simulink model "pid_board"  (R2024b)
settings: Solver=ode4  StartTime=0.0  StopTime=10.0  FixedStep=pcb.sim_dt  RelTol=1e-3
PostLoadFcn:
  | pbdir_ = fileparts(get_param('pid_board', 'FileName')); if ~exist('pcb', 'var'), run(fullfile(pbdir_, 'pid_board_params.m')); end; if ~exist('CtrlIn', 'var'), run(fullfile(pbdir_, '..', 'common', 'quad_ctrl_buses.m')); end; clear pbdir_
model workspace (MAT data in the model file):
  board_variant = Simulink.Parameter
  board_variant.Value = 1
  board_variant.Complexity = 'real'
  board_variant.Dimensions = [1 1]
  board_variant.Description = 'Analog section: 1 = pid_analog_fast, 2 = pid_analog_circuit'
  board_variant.DataType = 'double'
values from neighbouring files (symbols this model uses):
  pcb = evalin('base', 'pcb')    [pid_analog_circuit_test.m]    (also in pid_board_bench_inputs.m; pid_board_params.m = struct(); pid_board_validate.m)
Description:
  | PID_Board rev B digital twin (Model 2, fast). ctrl_in (CtrlIn bus) -> shim U1 -> DACs -> analog section (variant pcb.variant) -> control_io U3 -> esc_us [M1 RR, M2 FR, M3 RL, M4 FL].
settings Model: ParameterArgumentNames=board_variant  Creator=doubi  LastModifiedBy=doubi

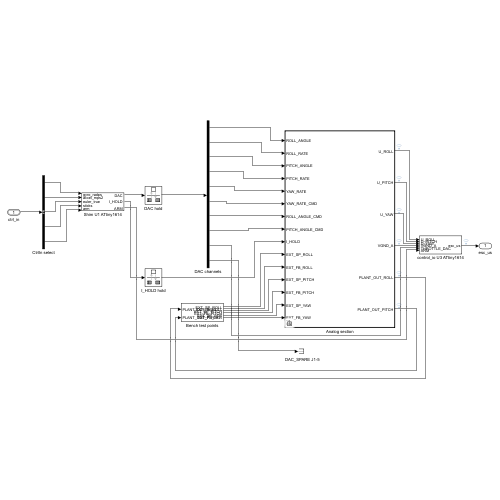
[thumbnail: Simulink's stored preview of the top-level diagram]
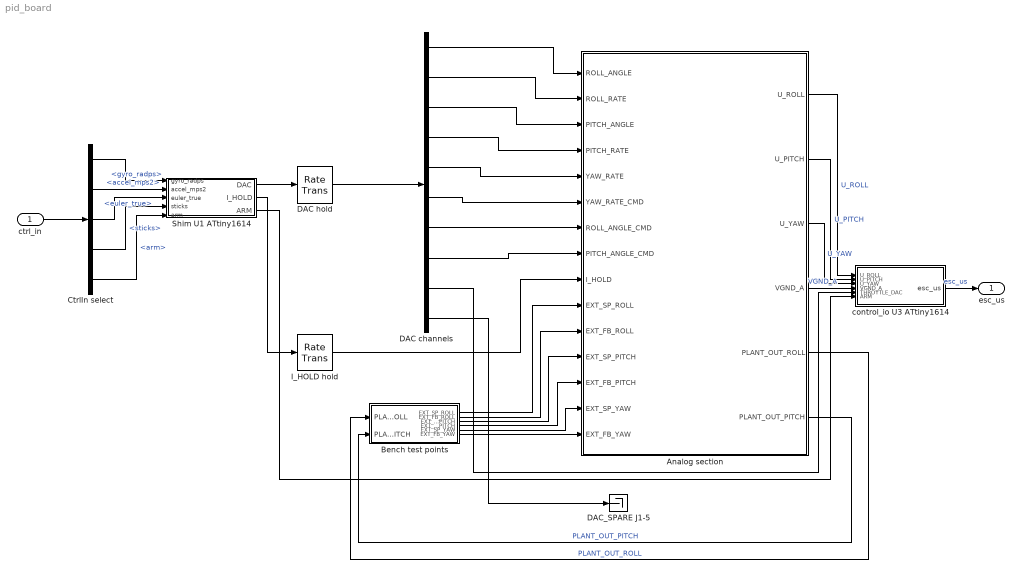
== system pid_board ==
  ctrl_in : Inport  OutDataTypeStr=Bus: CtrlIn  SampleTime=1e-3
  Analog section : Subsystem  Variant=on  VariantActivationTime=startup
  Bench test points : Subsystem  mask{brd=pcb}
      mask init:
      | w1p = [brd.VG + brd.bench.w1_offset, brd.bench.w1_amp, brd.bench.w1_freq, brd.bench.w1_t0];
  CtrlIn select : BusSelector  OutputSignals=gyro_radps,accel_mps2,euler_true,sticks,arm
  DAC channels : Demux  Outputs=10
  DAC hold : RateTransition  OutPortSampleTime=0
  DAC_SPARE J1-5 : Terminator
  I_HOLD hold : RateTransition  OutPortSampleTime=0
  Shim U1 ATtiny1614 : Subsystem  mask{brd=pcb}
      mask init:
      | Ts = brd.shim.Ts; g0 = 9.80665;
      | shp = [brd.shim.Ts, brd.shim.cf_alpha, brd.shim.axis_sign(:).', brd.shim.angle_src, brd.scale.Kw, brd.scale.Ktheta, brd.shim.angle_max, brd.shim.yaw_rate_max, brd.scale.thr_V0, brd.scale.thr_V1, brd.shim.ihold_low_thr, brd.shim.thr_low, brd.ihold.t_release, brd.VG];
      | crp = [brd.shim.crsf_min, brd.shim.crsf_mid, brd.shim.crsf_max];
      | nstd = brd.shim.noise_on*brd.shim.gyro_nd*sqrt(1/(2*brd.shim.Ts));
  control_io U3 ATtiny1614 : Subsystem  mask{brd=pcb}
      mask init:
      | Ts = brd.ctrl.Ts;
      | cp = [brd.ctrl.adc_lsb, brd.ctrl.adc_bits, brd.scale.thr_V0, brd.scale.thr_V1, brd.ctrl.us_off, brd.ctrl.us_idle, brd.ctrl.us_max, brd.ctrl.us_res, brd.ctrl.K_rpy(:).'];
      | mixm = brd.ctrl.mix;
  esc_us : Outport
  wires:
  ctrl_in/1 -> CtrlIn select/1
  CtrlIn select/2 -> Shim U1 ATtiny1614/2(accel_mps2)  "<accel_mps2>"
  CtrlIn select/4 -> Shim U1 ATtiny1614/4(sticks)  "<sticks>"
  Shim U1 ATtiny1614/2(I_HOLD) -> I_HOLD hold/1
  CtrlIn select/1 -> Shim U1 ATtiny1614/1(gyro_radps)  "<gyro_radps>"
  CtrlIn select/3 -> Shim U1 ATtiny1614/3(euler_true)  "<euler_true>"
  CtrlIn select/5 -> Shim U1 ATtiny1614/5(arm)  "<arm>"
  Bench test points/1(EXT_SP_ROLL) -> Analog section/10(EXT_SP_ROLL)
  Shim U1 ATtiny1614/1(DAC) -> DAC hold/1
  Shim U1 ATtiny1614/3(ARM) -> control_io U3 ATtiny1614/6(ARM)
  control_io U3 ATtiny1614/1(esc_us) -> esc_us/1  "esc_us"
  Analog section/4(VGND_A) -> control_io U3 ATtiny1614/4(VGND_A)  "VGND_A"
  DAC hold/1 -> DAC channels/1
  DAC channels/6 -> Analog section/6(YAW_RATE_CMD)
  I_HOLD hold/1 -> Analog section/9(I_HOLD)
  DAC channels/1 -> Analog section/1(ROLL_ANGLE)
  DAC channels/2 -> Analog section/2(ROLL_RATE)
  DAC channels/3 -> Analog section/3(PITCH_ANGLE)
  DAC channels/4 -> Analog section/4(PITCH_RATE)
  DAC channels/5 -> Analog section/5(YAW_RATE)
  DAC channels/7 -> Analog section/7(ROLL_ANGLE_CMD)
  Analog section/5(PLANT_OUT_ROLL) -> Bench test points/1(PLANT_OUT_ROLL)  "PLANT_OUT_ROLL"
  DAC channels/8 -> Analog section/8(PITCH_ANGLE_CMD)
  Analog section/6(PLANT_OUT_PITCH) -> Bench test points/2(PLANT_OUT_PITCH)  "PLANT_OUT_PITCH"
  DAC channels/9 -> control_io U3 ATtiny1614/5(THROTTLE_DAC)
  Analog section/3(U_YAW) -> control_io U3 ATtiny1614/3(U_YAW)  "U_YAW"
  DAC channels/10 -> DAC_SPARE J1-5/1
  Bench test points/2(EXT_FB_ROLL) -> Analog section/11(EXT_FB_ROLL)
  Bench test points/3(EXT_SP_PITCH) -> Analog section/12(EXT_SP_PITCH)
  Bench test points/4(EXT_FB_PITCH) -> Analog section/13(EXT_FB_PITCH)
  Bench test points/5(EXT_SP_YAW) -> Analog section/14(EXT_SP_YAW)
  Bench test points/6(EXT_FB_YAW) -> Analog section/15(EXT_FB_YAW)
  Analog section/1(U_ROLL) -> control_io U3 ATtiny1614/1(U_ROLL)  "U_ROLL"
  Analog section/2(U_PITCH) -> control_io U3 ATtiny1614/2(U_PITCH)  "U_PITCH"

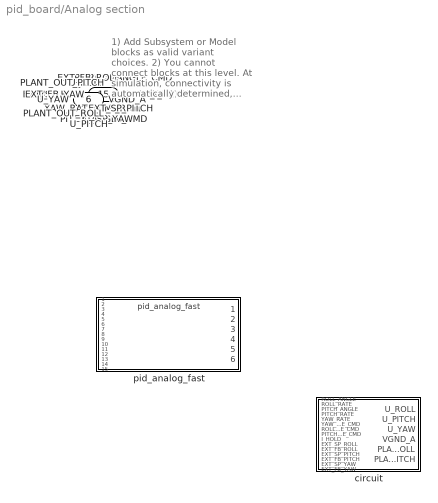
== system pid_board/Analog section ==
  note: 1) Add Subsystem or Model blocks as valid variant choices.
      | 2) You cannot connect blocks at this level. At simulation, connectivity is automatically
      | determined, based on the active variant and port name matching.
  ROLL_ANGLE : Inport
  ROLL_RATE : Inport  Port=2
  PITCH_ANGLE : Inport  Port=3
  PITCH_RATE : Inport  Port=4
  YAW_RATE : Inport  Port=5
  YAW_RATE_CMD : Inport  Port=6
  ROLL_ANGLE_CMD : Inport  Port=7
  PITCH_ANGLE_CMD : Inport  Port=8
  I_HOLD : Inport  Port=9
  EXT_SP_ROLL : Inport  Port=10
  EXT_FB_ROLL : Inport  Port=11
  EXT_SP_PITCH : Inport  Port=12
  EXT_FB_PITCH : Inport  Port=13
  EXT_SP_YAW : Inport  Port=14
  EXT_FB_YAW : Inport  Port=15
  circuit : Subsystem  TreatAsAtomicUnit=on  Variant=on  VariantControl=board_variant == 2  AllowZeroVariantControls=on
  pid_analog_fast : ModelReference  ModelNameDialog=pid_analog_fast  SimulationMode=Normal  VariantControl=board_variant == 1  ModelReferenceVersion=1.1
  U_ROLL : Outport
  U_PITCH : Outport  Port=2
  U_YAW : Outport  Port=3
  VGND_A : Outport  Port=4
  PLANT_OUT_ROLL : Outport  Port=5
  PLANT_OUT_PITCH : Outport  Port=6

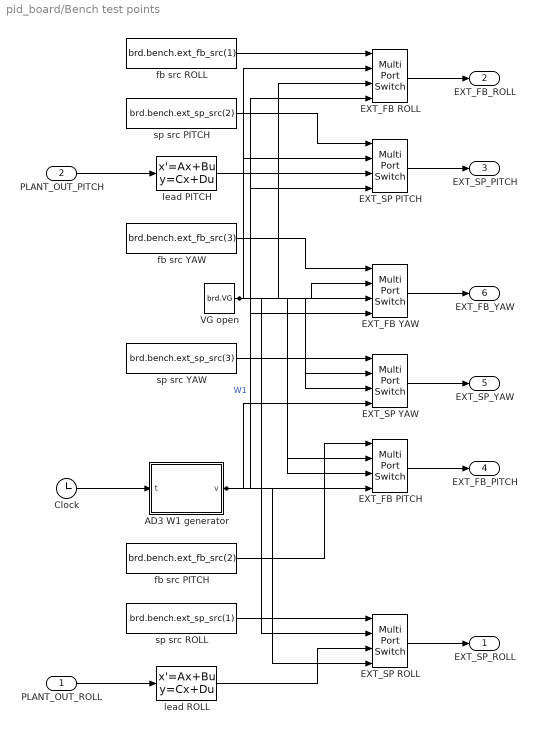
== system pid_board/Bench test points ==
  PLANT_OUT_ROLL : Inport
  PLANT_OUT_PITCH : Inport  Port=2
  AD3 W1 generator : MATLAB Function  TreatAsAtomicUnit=on
  Clock : Clock
  EXT_FB PITCH : MultiPortSwitch  DataPortOrder=Zero-based contiguous  zeroidx=on  SaturateOnIntegerOverflow=off  InputSameDT=off
  EXT_FB ROLL : MultiPortSwitch  DataPortOrder=Zero-based contiguous  zeroidx=on  SaturateOnIntegerOverflow=off  InputSameDT=off
  EXT_FB YAW : MultiPortSwitch  DataPortOrder=Zero-based contiguous  zeroidx=on  SaturateOnIntegerOverflow=off  InputSameDT=off
  EXT_SP PITCH : MultiPortSwitch  DataPortOrder=Zero-based contiguous  zeroidx=on  SaturateOnIntegerOverflow=off  InputSameDT=off
  EXT_SP ROLL : MultiPortSwitch  DataPortOrder=Zero-based contiguous  zeroidx=on  SaturateOnIntegerOverflow=off  InputSameDT=off
  EXT_SP YAW : MultiPortSwitch  DataPortOrder=Zero-based contiguous  zeroidx=on  SaturateOnIntegerOverflow=off  InputSameDT=off
  VG open : Constant  Value=brd.VG  SampleTime=0
  fb src PITCH : Constant  Value=brd.bench.ext_fb_src(2)
  fb src ROLL : Constant  Value=brd.bench.ext_fb_src(1)
  fb src YAW : Constant  Value=brd.bench.ext_fb_src(3)
  lead PITCH : StateSpace  A=-1/brd.bench.lead_tau  B=1/brd.bench.lead_tau  D=0  InitialCondition=brd.VG
  lead ROLL : StateSpace  A=-1/brd.bench.lead_tau  B=1/brd.bench.lead_tau  D=0  InitialCondition=brd.VG
  sp src PITCH : Constant  Value=brd.bench.ext_sp_src(2)
  sp src ROLL : Constant  Value=brd.bench.ext_sp_src(1)
  sp src YAW : Constant  Value=brd.bench.ext_sp_src(3)
  EXT_SP_ROLL : Outport
  EXT_FB_ROLL : Outport  Port=2
  EXT_SP_PITCH : Outport  Port=3
  EXT_FB_PITCH : Outport  Port=4
  EXT_SP_YAW : Outport  Port=5
  EXT_FB_YAW : Outport  Port=6
  wires:
  PLANT_OUT_PITCH/1 -> lead PITCH/1
  VG open/1 -> EXT_SP ROLL/2, EXT_FB ROLL/2, EXT_FB PITCH/2, EXT_FB ROLL/3, EXT_SP YAW/2, EXT_SP YAW/3, EXT_SP PITCH/2, EXT_FB YAW/2, EXT_FB PITCH/3, EXT_FB YAW/3
  Clock/1 -> AD3 W1 generator/1(t)
  PLANT_OUT_ROLL/1 -> lead ROLL/1
  lead PITCH/1 -> EXT_SP PITCH/3
  sp src PITCH/1 -> EXT_SP PITCH/1
  fb src ROLL/1 -> EXT_FB ROLL/1
  fb src YAW/1 -> EXT_FB YAW/1
  EXT_SP YAW/1 -> EXT_SP_YAW/1
  sp src YAW/1 -> EXT_SP YAW/1
  AD3 W1 generator/1(v) -> EXT_SP ROLL/4, EXT_FB ROLL/4, EXT_FB PITCH/4, EXT_SP PITCH/4, EXT_SP YAW/4, EXT_FB YAW/4  "W1"
  EXT_FB ROLL/1 -> EXT_FB_ROLL/1
  fb src PITCH/1 -> EXT_FB PITCH/1
  sp src ROLL/1 -> EXT_SP ROLL/1
  lead ROLL/1 -> EXT_SP ROLL/3
  EXT_SP PITCH/1 -> EXT_SP_PITCH/1
  EXT_FB YAW/1 -> EXT_FB_YAW/1
  EXT_FB PITCH/1 -> EXT_FB_PITCH/1
  EXT_SP ROLL/1 -> EXT_SP_ROLL/1

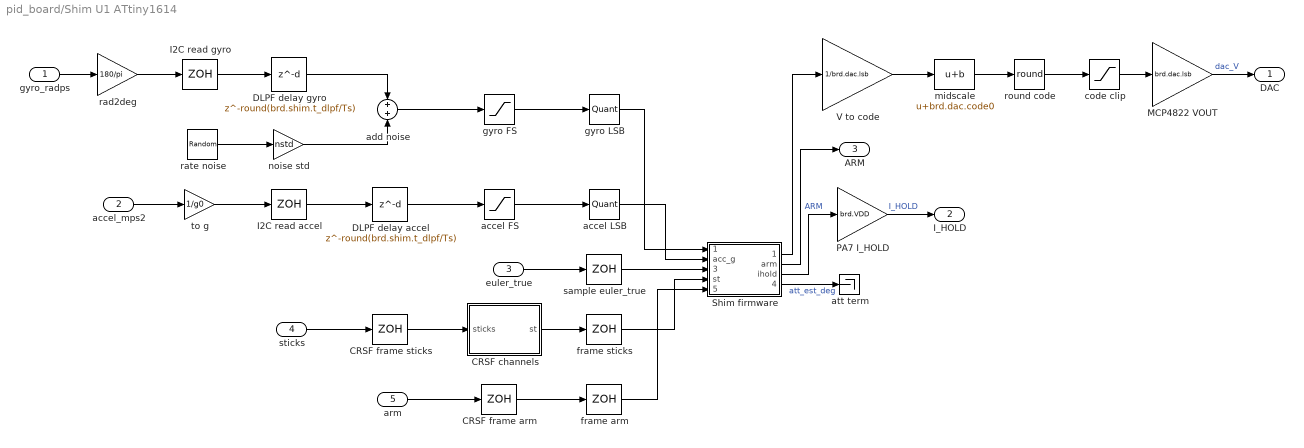
== system pid_board/Shim U1 ATtiny1614 ==
  gyro_radps : Inport
  accel_mps2 : Inport  Port=2
  euler_true : Inport  Port=3
  sticks : Inport  Port=4
  arm : Inport  Port=5
  CRSF channels : MATLAB Function  TreatAsAtomicUnit=on
  CRSF frame arm : ZeroOrderHold  SampleTime=brd.shim.crsf_Ts
  CRSF frame sticks : ZeroOrderHold  SampleTime=brd.shim.crsf_Ts
  DLPF delay accel : Delay  DelayLength=round(brd.shim.t_dlpf/Ts)
  DLPF delay gyro : Delay  DelayLength=round(brd.shim.t_dlpf/Ts)
  I2C read accel : ZeroOrderHold  SampleTime=Ts
  I2C read gyro : ZeroOrderHold  SampleTime=Ts
  MCP4822 VOUT : Gain  Gain=brd.dac.lsb
  PA7 I_HOLD : Gain  Gain=brd.VDD
  Shim firmware : MATLAB Function  TreatAsAtomicUnit=on
  V to code : Gain  Gain=1/brd.dac.lsb
  accel FS : Saturate  UpperLimit=brd.shim.acc_fs  LowerLimit=-brd.shim.acc_fs
  accel LSB : Quantizer  QuantizationInterval=brd.shim.acc_lsb
  add noise : Sum
  att term : Terminator
  code clip : Saturate  UpperLimit=2^brd.dac.bits - 1  LowerLimit=0
  frame arm : ZeroOrderHold  SampleTime=Ts
  frame sticks : ZeroOrderHold  SampleTime=Ts
  gyro FS : Saturate  UpperLimit=brd.shim.gyro_fs  LowerLimit=-brd.shim.gyro_fs
  gyro LSB : Quantizer  QuantizationInterval=brd.shim.gyro_lsb
  midscale : Bias  Bias=brd.dac.code0  SaturateOnIntegerOverflow=off
  noise std : Gain  Gain=nstd
  rad2deg : Gain  Gain=180/pi
  rate noise : RandomNumber  Mean=[0 0 0]  Variance=[1 1 1]  Seed=[23341 23342 23343]  SampleTime=Ts
  round code : Rounding  Operator=round
  sample euler_true : ZeroOrderHold  SampleTime=Ts
  to g : Gain  Gain=1/g0
  DAC : Outport
  I_HOLD : Outport  Port=2
  ARM : Outport  Port=3
  wires:
  gyro_radps/1 -> rad2deg/1
  noise std/1 -> add noise/2
  I2C read gyro/1 -> DLPF delay gyro/1
  rate noise/1 -> noise std/1
  frame arm/1 -> Shim firmware/5(arm_in)
  rad2deg/1 -> I2C read gyro/1
  euler_true/1 -> sample euler_true/1
  to g/1 -> I2C read accel/1
  accel FS/1 -> accel LSB/1
  accel_mps2/1 -> to g/1
  frame sticks/1 -> Shim firmware/4(st)
  DLPF delay gyro/1 -> add noise/1
  I2C read accel/1 -> DLPF delay accel/1
  sticks/1 -> CRSF frame sticks/1
  add noise/1 -> gyro FS/1
  PA7 I_HOLD/1 -> I_HOLD/1  "I_HOLD"
  accel LSB/1 -> Shim firmware/2(acc_g)
  DLPF delay accel/1 -> accel FS/1
  sample euler_true/1 -> Shim firmware/3(euler_rad)
  CRSF frame sticks/1 -> CRSF channels/1(sticks)
  arm/1 -> CRSF frame arm/1
  gyro FS/1 -> gyro LSB/1
  CRSF channels/1(st) -> frame sticks/1
  CRSF frame arm/1 -> frame arm/1
  gyro LSB/1 -> Shim firmware/1(gyro_dps)
  Shim firmware/1(dac_rel) -> V to code/1
  Shim firmware/2(arm) -> ARM/1  "ARM"
  midscale/1 -> round code/1
  Shim firmware/3(ihold) -> PA7 I_HOLD/1
  Shim firmware/4(att_deg) -> att term/1  "att_est_deg"
  V to code/1 -> midscale/1
  round code/1 -> code clip/1
  code clip/1 -> MCP4822 VOUT/1
  MCP4822 VOUT/1 -> DAC/1  "dac_V"

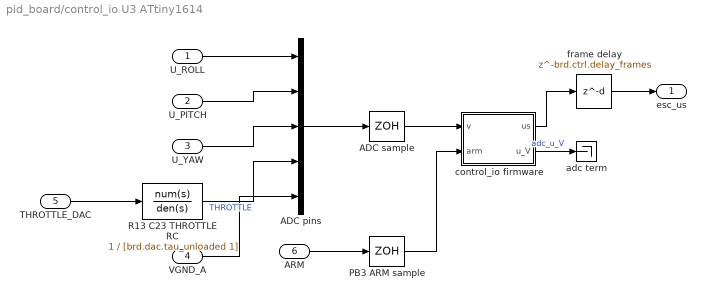
== system pid_board/control_io U3 ATtiny1614 ==
  U_ROLL : Inport
  U_PITCH : Inport  Port=2
  U_YAW : Inport  Port=3
  VGND_A : Inport  Port=4
  THROTTLE_DAC : Inport  Port=5
  ARM : Inport  Port=6
  ADC pins : Mux  Inputs=5
  ADC sample : ZeroOrderHold  SampleTime=Ts
  PB3 ARM sample : ZeroOrderHold  SampleTime=Ts
  R13 C23 THROTTLE RC : TransferFcn  Numerator=1  Denominator=[brd.dac.tau_unloaded 1]
  adc term : Terminator
  control_io firmware : MATLAB Function  TreatAsAtomicUnit=on
  frame delay : Delay  DelayLength=brd.ctrl.delay_frames  InitialCondition=brd.ctrl.us_off
  esc_us : Outport
  wires:
  U_YAW/1 -> ADC pins/3
  THROTTLE_DAC/1 -> R13 C23 THROTTLE RC/1
  U_ROLL/1 -> ADC pins/1
  ARM/1 -> PB3 ARM sample/1
  ADC pins/1 -> ADC sample/1
  R13 C23 THROTTLE RC/1 -> ADC pins/4  "THROTTLE"
  VGND_A/1 -> ADC pins/5
  U_PITCH/1 -> ADC pins/2
  ADC sample/1 -> control_io firmware/1(v)
  control_io firmware/1(us) -> frame delay/1
  PB3 ARM sample/1 -> control_io firmware/2(arm)
  control_io firmware/2(u_V) -> adc term/1  "adc_u_V"
  frame delay/1 -> esc_us/1

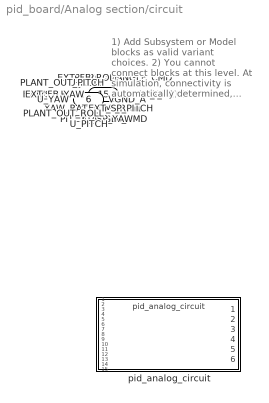
== system pid_board/Analog section/circuit ==
  note: 1) Add Subsystem or Model blocks as valid variant choices.
      | 2) You cannot connect blocks at this level. At simulation, connectivity is automatically
      | determined, based on the active variant and port name matching.
  ROLL_ANGLE : Inport
  ROLL_RATE : Inport  Port=2
  PITCH_ANGLE : Inport  Port=3
  PITCH_RATE : Inport  Port=4
  YAW_RATE : Inport  Port=5
  YAW_RATE_CMD : Inport  Port=6
  ROLL_ANGLE_CMD : Inport  Port=7
  PITCH_ANGLE_CMD : Inport  Port=8
  I_HOLD : Inport  Port=9
  EXT_SP_ROLL : Inport  Port=10
  EXT_FB_ROLL : Inport  Port=11
  EXT_SP_PITCH : Inport  Port=12
  EXT_FB_PITCH : Inport  Port=13
  EXT_SP_YAW : Inport  Port=14
  EXT_FB_YAW : Inport  Port=15
  pid_analog_circuit : ModelReference  ModelNameDialog=pid_analog_circuit  SimulationMode=Normal  VariantControl=pcb.circuit_enable == 1  ModelReferenceVersion=1.10
  U_ROLL : Outport
  U_PITCH : Outport  Port=2
  U_YAW : Outport  Port=3
  VGND_A : Outport  Port=4
  PLANT_OUT_ROLL : Outport  Port=5
  PLANT_OUT_PITCH : Outport  Port=6

== matlab function pid_board/Shim U1 ATtiny1614/Shim firmware ==
  data: gyro_dps input size=[3 1]; dac_rel output size=[10 1]; acc_g input size=[3 1]; euler_rad input size=[3 1]; st input size=[4 1]; arm_in input size=1; arm output size=1; ihold output size=1; att_deg output size=[2 1]; shp parameter
function [dac_rel, arm, ihold, att_deg] = shim_fw(gyro_dps, acc_g, euler_rad, st, arm_in, shp)
%Shim U1 firmware model (ASSUMED behaviour, no PCB firmware exists).
% shp = [Ts alpha sgn_r sgn_p sgn_y angle_src Kw Kth angle_max yaw_max thr_V0 thr_V1
%        ihold_low thr_low t_release VG]
% dac_rel: 10 DAC channels in pcb.dac.order, volts relative to VG.
persistent phi th k init
Ts = shp(1); a = shp(2); sg = shp(3:5); Kw = shp(7); Kth = shp(8);
if isempty(k)
    k = 0; phi = 0; th = 0; init = false;
end
% accelerometer tilt (specific force, FRD): phi = atan2(-fy,-fz), theta = atan2(fx, |fyz|)
phi_a = atan2(-acc_g(2), -acc_g(3))*180/pi;
th_a = atan2(acc_g(1), sqrt(acc_g(2)^2 + acc_g(3)^2))*180/pi;
if ~init  % seed from the accelerometer at boot (first valid sample after the DLPF delay)
    phi = phi_a; th = th_a;
    init = norm(acc_g) > 0.5;
else
    phi = a*(phi + gyro_dps(1)*Ts) + (1 - a)*phi_a;
    th = a*(th + gyro_dps(2)*Ts) + (1 - a)*th_a;
end
if shp(6) > 0.5
    ang = [phi; th];
else
    ang = euler_rad(1:2)*180/pi;
end
thr = min(max(st(4), 0), 1);
dac_rel = zeros(10, 1);
dac_rel(1) = Kth*sg(1)*ang(1);                 % ROLL_ANGLE
dac_rel(2) = Kw*sg(1)*gyro_dps(1);             % ROLL_RATE
dac_rel(3) = Kth*sg(2)*ang(2);                 % PITCH_ANGLE
dac_rel(4) = Kw*sg(2)*gyro_dps(2);             % PITCH_RATE
dac_rel(5) = Kw*sg(3)*gyro_dps(3);             % YAW_RATE
dac_rel(6) = Kw*sg(3)*shp(10)*st(3);           % YAW_RATE_CMD   (yaw +1 = nose right)
dac_rel(7) = Kth*sg(1)*shp(9)*st(1);           % ROLL_ANGLE_CMD (roll +1 = phi > 0)
dac_rel(8) = Kth*sg(2)*(-shp(9)*st(2));        % PITCH_ANGLE_CMD (pitch +1 = nose down = theta < 0)
dac_rel(9) = shp(11) + thr*(shp(12) - shp(11)) - shp(16);  % THROTTLE (absolute scale)
dac_rel(10) = 0;                               % DAC_SPARE
armed = arm_in > 0.5;
arm = double(armed);
ihold = double(~armed || (shp(13) > 0.5 && thr < shp(14)) || k*Ts < shp(15));
att_deg = [phi; th];
k = k + 1;

== matlab function pid_board/Shim U1 ATtiny1614/CRSF channels ==
  data: sticks input size=[4 1]; st output size=[4 1]; crp parameter
function st = crsf(sticks, crp)
%ELRS -> CRSF 11-bit channels (172..992..1811) and back to normalised sticks
half = (crp(3) - crp(1))/2;
ch = zeros(4, 1);
ch(1:3) = round(crp(2) + sticks(1:3)*half);
ch(4) = round(crp(1) + sticks(4)*(crp(3) - crp(1)));
ch = min(max(ch, crp(1)), crp(3));
st = zeros(4, 1);
st(1:3) = (ch(1:3) - crp(2))/half;
st(4) = (ch(4) - crp(1))/(crp(3) - crp(1));

== matlab function pid_board/Bench test points/AD3 W1 generator ==
  data: t input size=1; v output size=1; w1p parameter
function v = w1(t, w1p)
%AD3 W1 generator: w1p = [level_abs amp freq t0]; freq 0 = step
v = w1p(1);
if t >= w1p(4)
    if w1p(3) > 0
        v = w1p(1) + w1p(2)*sin(2*pi*w1p(3)*(t - w1p(4)));
    else
        v = w1p(1) + w1p(2);
    end
end

== matlab function pid_board/control_io U3 ATtiny1614/control_io firmware ==
  data: v input size=[5 1]; us output size=[4 1]; arm input size=1; u_V output size=[3 1]; cp parameter; mixm parameter
function [us, u_V] = ctrl_fw(v, arm, cp, mixm)
%control_io U3 firmware model (ASSUMED): 10-bit ADC (VDD ref), quad-X mix, PWM 1000-2000 us
% v = [U_ROLL U_PITCH U_YAW THROTTLE VGND_A] absolute volts
% cp = [lsb bits thr_V0 thr_V1 us_off us_idle us_max us_res K_roll K_pitch K_yaw]
code = min(max(floor(v/cp(1)), 0), 2^cp(2) - 1);
vq = code*cp(1);
u_V = vq(1:3) - vq(5);
thr = min(max((vq(4) - cp(3))/(cp(4) - cp(3)), 0), 1);
thr_us = cp(5) + thr*(cp(7) - cp(5));
Krpy = [cp(9); cp(10); cp(11)];
m = mixm(:, 1)*thr_us + mixm(:, 2:4)*(Krpy.*u_V);
if arm > 0.5
    m = min(max(m, cp(6)), cp(7));
else
    m = cp(5)*ones(4, 1);
end
us = round(m/cp(8))*cp(8);
